simulink model "virtual_aero2_system_block_diagram"  (R2026a)
settings: Solver=ode1  StopTime=30  FixedStep=0.002
values from neighbouring files (symbols this model uses):
  Jeq = Jr + Jprop + Jh    (= 4.4030375e-05)    [aero2_parameters.m]
  Jp = 0.0231    [aero2_parameters.m]
  kd = 8*10^(-5)    (= 8e-05)    [aero2_parameters.m]
  km = 4.2*10^(-2)    (= 0.042)    [aero2_parameters.m]
  kt = 4.2*10^(-2)    (= 0.042)    [aero2_parameters.m]
  Rm = 8.4    [aero2_parameters.m]
undefined symbols (not defined in the file or in its folder): HIL, qc_get_step_size
libraries: quarc_library x3
settings Model: Creator=MLevis  LastModifiedBy=MLevis

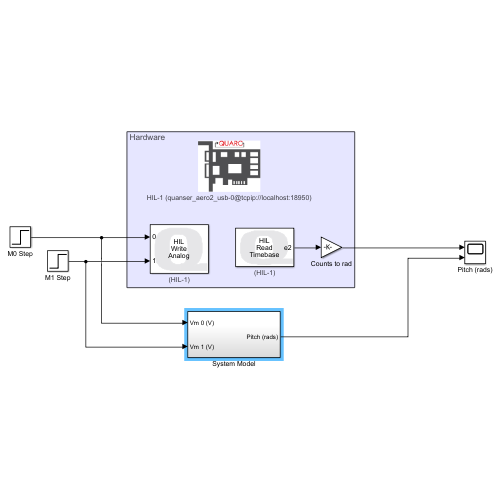
[thumbnail: Simulink's stored preview of the top-level diagram]
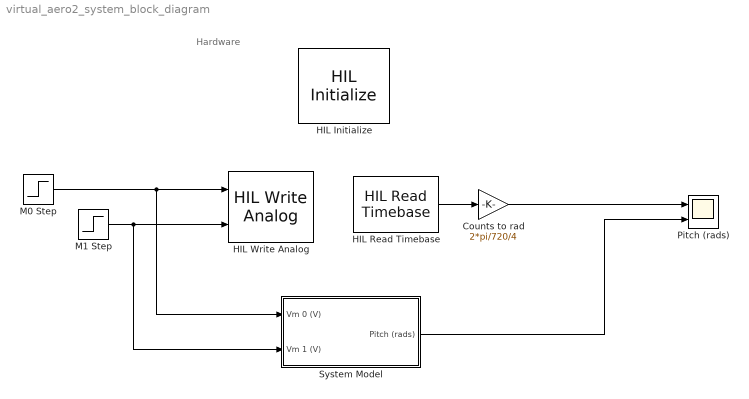
== system virtual_aero2_system_block_diagram ==
  note: Hardware
  Counts to rad : Gain  Gain=2*pi/720/4
  HIL Initialize : quarc_library/Data Acquisition/Generic/Configuration/HIL Initialize  Priority=-99  object_name=HIL-1  board_type=quanser_aero2_usb  board_number=0@tcpip://localhost:18950  board_options=""  exclusive=off  active=on  hardware_clocks=[0]  clock_modes=[]  initial_clock_frequencies=[]  set_clock_params_at_start=off  set_clock_params_at_switch_in=off  set_clock_frequencies_at_start=off  set_clock_frequencies_at_switch_in=off  analog_input_channels=[0:1]  analog_input_configurations=[]  analog_input_maximums=3  analog_input_minimums=-3  set_analog_input_params_at_start=off  set_analog_input_params_at_switch_in=off  analog_output_channels=[0:1]  analog_output_maximums=24  analog_output_minimums=-24  initial_analog_outputs=[0]  final_analog_outputs=[0]  watchdog_analog_outputs=[0]  set_analog_output_params_at_start=off  set_analog_output_params_at_switch_in=off  set_analog_outputs_at_start=on  set_analog_outputs_at_switch_in=off  set_analog_outputs_at_terminate=on  set_analog_outputs_at_switch_out=off  set_analog_outputs_on_watchdog=on  digital_input_channels=[]  digital_output_channels=[0:1]  digital_output_configuration=[]  initial_digital_outputs=[1]  final_digital_outputs=[0]  watchdog_digital_outputs=[0]  set_digital_output_params_at_start=off  set_digital_output_params_at_switch_in=off  set_digital_outputs_at_start=on  set_digital_outputs_at_switch_in=off  set_digital_outputs_at_terminate=on  set_digital_outputs_at_switch_out=off  set_digital_outputs_on_watchdog=on  encoder_channels=[0:3]  quadrature=[4]  encoder_filter_frequency=[]  initial_encoder_counts=[0]  set_encoder_params_at_start=off  set_encoder_params_at_switch_in=off  set_encoder_counts_at_start=on  set_encoder_counts_at_switch_in=off  pwm_channels=[]  pwm_modes=[]  pwm_frequency=[]  pwm_configuration=[]  pwm_alignment=[]  pwm_polarity=[]  pwm_leading_deadband=[]  pwm_trailing_deadband=[]  initial_pwm_outputs=[]  final_pwm_outputs=[]  watchdog_pwm_outputs=[]  set_pwm_params_at_start=off  set_pwm_params_at_switch_in=off  set_pwm_outputs_at_start=off  set_pwm_outputs_at_switch_in=off  set_pwm_outputs_at_terminate=off  set_pwm_outputs_at_switch_out=off  set_pwm_outputs_on_watchdog=off  other_output_channels=[11000:11002]  initial_other_outputs=[0 1 0]  final_other_outputs=[1 0 0]  watchdog_other_outputs=[0 0 1]  set_other_outputs_at_start=on  set_other_outputs_at_switch_in=off  set_other_outputs_at_terminate=on  set_other_outputs_at_switch_out=off  set_other_outputs_on_watchdog=on
  HIL Read Timebase : quarc_library/Data Acquisition/Generic/Timebases/HIL Read Timebase  object_name=HIL-1  clock=0  analog_channels=[]  encoder_channels=[2]  digital_channels=[]  other_channels=[]  active=on  vector_output=off  port_labels=channel numbers  data_type_mode=Inherit via back propagation  encoder_data_type=double  digital_data_type=boolean  overflow_mode=Synchronize (for simulated cards only)  samples_in_buffer=max(ceil(1/qc_get_step_size), 1)
  HIL Write Analog : quarc_library/Data Acquisition/Generic/Immediate I//O/HIL Write Analog  object_name=HIL-1  channels=[0:1]  sample_time=-1  active=on  vector_input=off  port_labels=channel numbers
  M0 Step : Step  FinalValue=5  SampleTime=0
  M1 Step : Step  Time=5  FinalValue=5  SampleTime=0
  Pitch (rads) : Scope  NumInputPorts=2
      settings: ActiveDisplayYMinimum=-0.3521  ActiveDisplayYMaximum=0.74453
  System Model : Subsystem
  wires:
  M0 Step/1 -> System Model/1(Vm 0 (V)), HIL Write Analog/1
  Counts to rad/1 -> Pitch (rads)/1
  M1 Step/1 -> System Model/2(Vm 1 (V)), HIL Write Analog/2
  HIL Read Timebase/1 -> Counts to rad/1
  System Model/1(Pitch (rads)) -> Pitch (rads)/2

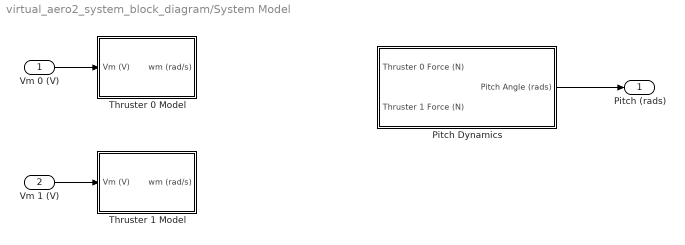
== system virtual_aero2_system_block_diagram/System Model ==
  Vm 0 (V) : Inport
  Vm 1 (V) : Inport  Port=2
  Pitch Dynamics : Subsystem
  Thruster 0 Model : Subsystem
  Thruster 1 Model : Subsystem
  Pitch (rads) : Outport
  wires:
  Vm 0 (V)/1 -> Thruster 0 Model/1(Vm (V))
  Vm 1 (V)/1 -> Thruster 1 Model/1(Vm (V))
  Pitch Dynamics/1(Pitch Angle (rads)) -> Pitch (rads)/1

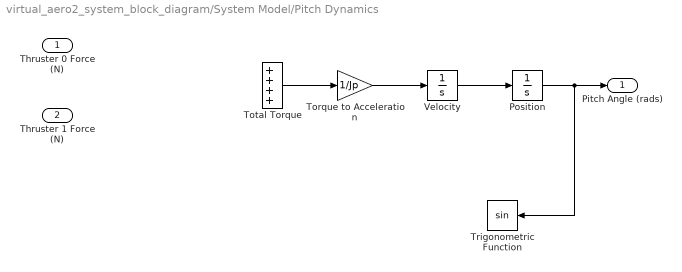
== system virtual_aero2_system_block_diagram/System Model/Pitch Dynamics ==
  Thruster 0 Force (N) : Inport
  Thruster 1 Force (N) : Inport  Port=2
  Position : Integrator
  Torque to Acceleration : Gain  Gain=1/Jp
  Total Torque : Sum  Inputs=++++
  Trigonometric Function : Trigonometry
  Velocity : Integrator
  Pitch Angle (rads) : Outport
  wires:
  Position/1 -> Trigonometric Function/1, Pitch Angle (rads)/1
  Torque to Acceleration/1 -> Velocity/1
  Velocity/1 -> Position/1
  Total Torque/1 -> Torque to Acceleration/1

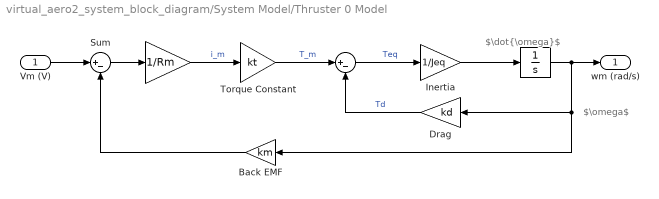
== system virtual_aero2_system_block_diagram/System Model/Thruster 0 Model ==
  note: $\omega$
  note: $\dot{\omega}$
  Vm (V) : Inport
  " " : Integrator
  "  " : Gain  Gain=1/Rm  SaturateOnIntegerOverflow=on  OutDataTypeStr=Inherit: Same as input  ParamDataTypeStr=Inherit: Same as input
  "   " : Sum  Inputs=|+-
  Back EMF : Gain  Gain=km
  Drag : Gain  Gain=kd
  Inertia : Gain  Gain=1/Jeq
  Sum : Sum  Inputs=|+-  InputSameDT=on  SaturateOnIntegerOverflow=on  OutDataTypeStr=Inherit: Same as first input
  Torque Constant : Gain  Gain=kt
  wm (rad/s) : Outport
  wires:
  "  "/1 -> Torque Constant/1  "i_m"
  Vm (V)/1 -> Sum/1
  Sum/1 -> "  "/1
  Back EMF/1 -> Sum/2
  Torque Constant/1 -> "   "/1  "T_m"
  "   "/1 -> Inertia/1  "Teq"
  Inertia/1 -> " "/1
  " "/1 -> Drag/1, Back EMF/1, wm (rad/s)/1
  Drag/1 -> "   "/2  "Td"

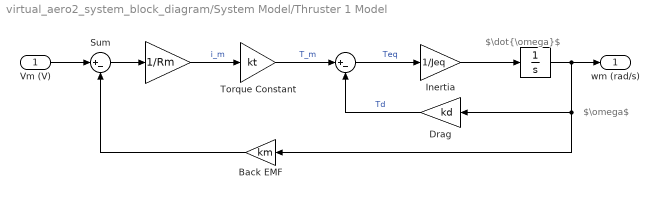
== system virtual_aero2_system_block_diagram/System Model/Thruster 1 Model ==
  note: $\dot{\omega}$
  note: $\omega$
  Vm (V) : Inport
  " " : Integrator
  "  " : Gain  Gain=1/Rm  SaturateOnIntegerOverflow=on  OutDataTypeStr=Inherit: Same as input  ParamDataTypeStr=Inherit: Same as input
  "   " : Sum  Inputs=|+-
  Back EMF : Gain  Gain=km
  Drag : Gain  Gain=kd
  Inertia : Gain  Gain=1/Jeq
  Sum : Sum  Inputs=|+-  InputSameDT=on  SaturateOnIntegerOverflow=on  OutDataTypeStr=Inherit: Same as first input
  Torque Constant : Gain  Gain=kt
  wm (rad/s) : Outport
  wires:
  Drag/1 -> "   "/2  "Td"
  " "/1 -> wm (rad/s)/1, Back EMF/1, Drag/1
  Inertia/1 -> " "/1
  "   "/1 -> Inertia/1  "Teq"
  Torque Constant/1 -> "   "/1  "T_m"
  Back EMF/1 -> Sum/2
  Sum/1 -> "  "/1
  Vm (V)/1 -> Sum/1
  "  "/1 -> Torque Constant/1  "i_m"
